simulink model "carsim_with_simulink14dof_random_control"  (R2023b)
settings: Solver=FixedStepAuto  StartTime=0.0  StopTime=25  FixedStep=0.001  RelTol=1e-3  EnableMultiTasking=on
values from neighbouring files (symbols this model uses):
  A = 5    [unlinear_vehicle_Parameters.m]
  Bf = 1.725    [unlinear_vehicle_Parameters.m]
  Br = 1.750    (= 1.75)    [unlinear_vehicle_Parameters.m]
  Cd = 0.4    [unlinear_vehicle_Parameters.m]
  Cs_f = 4302    [unlinear_vehicle_Parameters.m]
  f = 0.01    [unlinear_vehicle_Parameters.m]
  g = 9.8    [Truck_simulate.m]    (also in unlinear_vehicle_Parameters.m)
  He = 0.45    [unlinear_vehicle_Parameters.m]
  Hp = 0.2    [unlinear_vehicle_Parameters.m]
  I_tire = 0.7    [unlinear_vehicle_Parameters.m]
  Ix = 423.3    [unlinear_vehicle_Parameters.m]
  Iy = 1762.5    [unlinear_vehicle_Parameters.m]
  Iz = 1762.5    [unlinear_vehicle_Parameters.m]
  ks_f = 189000    [unlinear_vehicle_Parameters.m]
  kw = 220000    [unlinear_vehicle_Parameters.m]
  Lf = 1.330    (= 1.33)    [unlinear_vehicle_Parameters.m]
  Lr = 3.140 - 1.330    (= 1.81)    [unlinear_vehicle_Parameters.m]
  m = m_sprung + m_load + m_unsprung    (= 10505)    [Truck_simulate.m]    (also in unlinear_vehicle_Parameters.m = 1407.3)
  mb = 1128.5 + 000    (= 1128.5)    [unlinear_vehicle_Parameters.m]
  mw = 139.4 / 2    (= 69.7)    [unlinear_vehicle_Parameters.m]
  p = 1.206    [unlinear_vehicle_Parameters.m]
  r = 0.510    (= 0.51)    [Truck_simulate.m]    (also in unlinear_vehicle_Parameters.m = 0.287)
  vx0 = 5    [Truck_simulate.m]    (also in unlinear_vehicle_Parameters.m)
  vy0 = 0    [Truck_simulate.m]    (also in unlinear_vehicle_Parameters.m)
  w0 = vx0 / r    (= 9.80392156863)    [Truck_simulate.m]    (also in unlinear_vehicle_Parameters.m = 17.4216027875)
  wz0 = 0    [Truck_simulate.m]    (also in unlinear_vehicle_Parameters.m)
undefined symbols (not defined in the file or in its folder): Delta_act_seed, T_motor_seed
libraries: cstblocks x2, Solver_SF x1
(part 1 of 2)
settings Model: Creator=dzY  LastModifiedBy=Admin
settings SolverCC: AlgebraicLoopSolver=TrustRegion
settings DataIOCC: SaveFormat=Array  ReturnWorkspaceOutputs=off
settings OptimizationCC: LifeSpan=inf
settings DebuggingCC: SolverPrmCheckMsg=warning  UnconnectedInputMsg=warning  UnconnectedOutputMsg=warning  UnconnectedLineMsg=warning  SFUnexpectedBacktrackingDiag=warning  SFNoUnconditionalDefaultTransitionDiag=warning  SFExecutionAtInitializationDiag=none  ArithmeticOperatorsInVariantConditions=warning
settings HardwareCC: ProdBitPerPointer=32  ProdBitPerSizeT=32  ProdBitPerPtrDiffT=32  ProdLargestAtomicFloat=None  ProdIntDivRoundTo=Undefined  ProdEndianess=Unspecified  ProdWordSize=32  ProdHWDeviceType=32-bit Generic
settings ModelReferenceCC: EnableRefExpFcnMdlSchedulingChecks=on  PropagateSignalLabelsOutOfModel=off
settings SFSimCC: SimUseLocalCustomCode=off  CustomCodeUndefinedFunction=UseInterfaceOnly
settings RTWCC: RTWUseLocalCustomCode=off
settings CodeAppCC: StateflowObjectComments=on
settings GRTTargetCC: TargetLangStandard=C89/C90 (ANSI)
settings ConfigComp: CovMetricSettings=dw  CovSaveCumulativeToWorkspaceVar=on  CovSaveSingleToWorkspaceVar=on  CovExternalEMLEnable=off  CovSFcnEnable=off

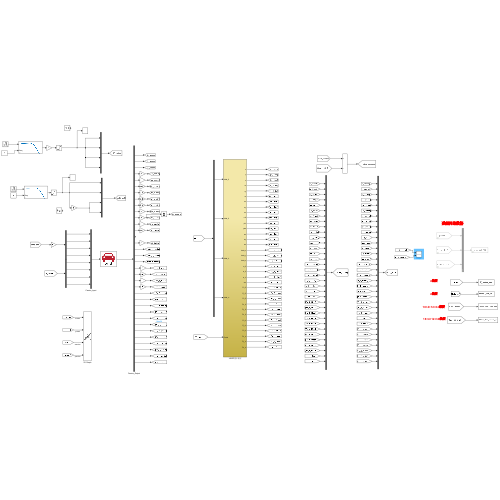
[thumbnail: Simulink's stored preview of the top-level diagram]
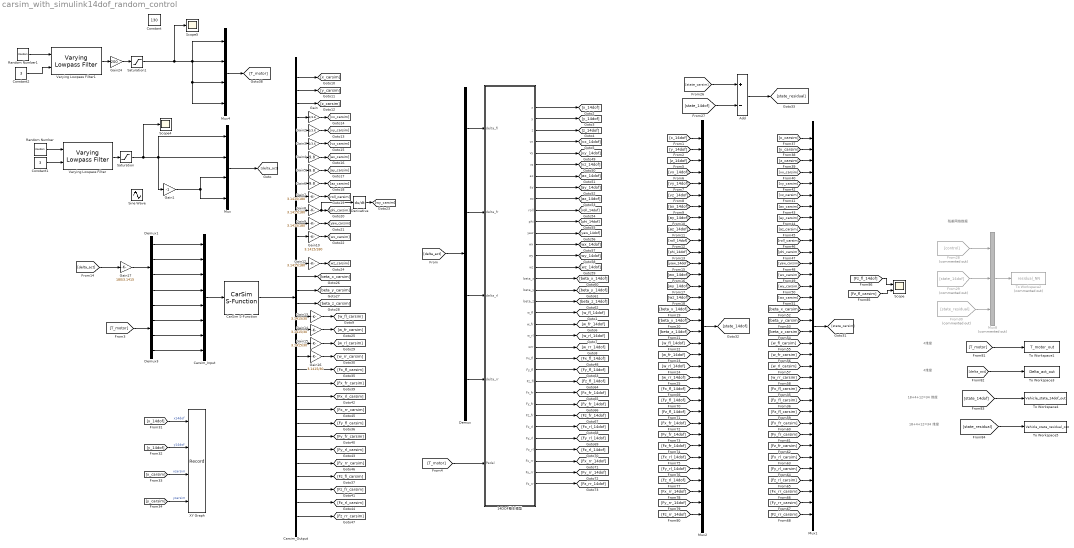
== system carsim_with_simulink14dof_random_control ==
  note: 4维度
  note: 残差网络数据
  note: 4维度
  note: 18+4+12=34维度
  note: 18+4+12=34维度
  14DOF整车模型 : Subsystem
  Add : Sum  Inputs=+-
  CarSim S-Function : Solver_SF/CarSim S-Function  Priority=1  SIMFILE=simfile.sim  Run_RTs=off  vs_state_ind=Run  StopMode_ind=Vehicle Model
  Carsim_Input : Mux  Inputs=8
  Carsim_Output : Demux  Outputs=34
  Constant : Constant  Value=130
  Constant1 : Constant  Value=3
  Constant2 : Constant  Value=3
  Demux : Demux
  Demux1 : Demux
  Demux3 : Demux
  Derivative : Derivative
  From28 : From  Commented=on  GotoTag=control
  From29 : From  Commented=on  GotoTag=state_14dof
  From30 : From  Commented=on  GotoTag=state_residual
  Gain : Gain  Gain=1/3.6
  Gain1 : Gain  Gain=-1
  Gain{7..10,12} (5 alike) : Gain  Gain=3.1415/180
  Gain{13..16} (4 alike) : Gain  Gain=3.1415/30
  Gain17 : Gain  Gain=180/3.1415
  Gain2 : Gain  Gain=1/3.6
  Gain24 : Gain  Gain=200
  Gain3 : Gain  Gain=1/3.6
  Gain4 : Gain  Gain=9.8
  Gain5 : Gain  Gain=9.8
  Gain6 : Gain  Gain=9.8
  Mux : Mux
  Mux1 : Mux  Inputs=34
  Mux2 : Mux  Inputs=34
  Mux4 : Mux
  Mux8 : Mux  Commented=on  Inputs=3
  Random Number : RandomNumber  Variance=20  Seed=Delta_act_seed  SampleTime=0.001
  Random Number1 : RandomNumber  Mean=0.1  Variance=50  Seed=T_motor_seed  SampleTime=0.001
  Saturation : Saturate  UpperLimit=0.35  LowerLimit=-0.35
  Saturation1 : Saturate  UpperLimit=150  LowerLimit=-150
  Scope : Scope  NumInputPorts=2
  Scope4 : Scope
  Scope5 : Scope
  Sine Wave : Sin  Amplitude=0.25  Frequency=0.4  SampleTime=0
  To Workspace1 : ToWorkspace  VariableName=T_motor_out  SaveFormat=Timeseries  SampleTime=-1
  To Workspace2 : ToWorkspace  Commented=on  VariableName=residual_NN  SaveFormat=Timeseries  SampleTime=-1
  To Workspace3 : ToWorkspace  VariableName=Delta_act_out  SaveFormat=Timeseries  SampleTime=-1
  To Workspace4 : ToWorkspace  VariableName=Vehicle_state_14dof_out  SaveFormat=Timeseries  SampleTime=-1
  To Workspace5 : ToWorkspace  VariableName=Vehicle_state_residual_out  SaveFormat=Timeseries  SampleTime=-1
  Varying Lowpass Filter : cstblocks/Linear Parameter Varying/Varying Lowpass Filter  N=8
  Varying Lowpass Filter1 : cstblocks/Linear Parameter Varying/Varying Lowpass Filter  N=8
  XY Graph : Record  RecordToFile=on  FileSettingsInternal="{\"entries\":[{\"content\":{\"excelSettings\":{\"content\":{},\"type\":\"Streamout.ExcelSettings\"}},\"type\":\"Streamout.FileSettingStorage\",\"uuid\":\"\"}],\"packageUris\":[\"http:\\/\\/schema.mathworks.com\\/mf0\\/streamout_blocks\\/R2020a\"],\"version\":\"1.0\"}"  Layout=[1 1]  SignalsInternal="{\"entries\":[{\"content\":{\"signals\":[{\"content\":{\"blockPath\":[],\"dimensions\":[1],\"domain\":\"\",\"lineColor\":\"#a2142f\",\"plots\":[1],\"port\":1,\"sid\":[\"\"],\"signalID\":3004,\"signalName\":\"x14dof\"},\"type\":\"RecordBlkView.Signal\",\"uuid\":\"\"},{\"content\":{\"blockPath\":[],\"dimensions\":[1],\"domain\":\"\",\"lineColor\":\"#139fff\",\"plots\":[1],\"port\":2,\"sid\":[\"\"],\"signalID\":3008,\"signalName\":\"y14dof\"},\"type\":\"RecordBlkView.Signal\",\"uuid\":\"\"},{\"content\":{\"blockPath\":[],\"dimensions\":[1],\"domain\":\"\",\"lineColor\":\"#77ac30\",\"plots\":[1],\"port\":3,\"sid\":[\"\"],\"signalID\":3012,\"signalName\":\"xcarsim\"},\"type\":\"RecordBlkView.Signal\",\"uuid\":\"\"},{\"content\":{\"blockPath\":[],\"dimensions\":[1],\"domain\":\"\",\"lineColor\":\"#4dbeee\",\"plots\":[1],\"port\":4,\"sid\":[\"\"],\"signalID\":3016,\"signalName\":\"ycarsim\"},\"type\":\"RecordBlkView.Signal\",\"uuid\":\"\"}]},\"type\":\"RecordBlkView.InputSignals\",\"uuid\":\"\"}],\"packageUris\":[\"http:\\/\\/schema.mathworks.com\\/mf0\\/streamout_blocks\\/R2020a\"],\"version\":\"1.0\"}"  VisualizationBindings="{\"xyplotplugin\":{\"info\":[{\"series\":[{\"bindingParametersList\":[{\"parameter\":\"X-Axis\",\"signalID\":3004,\"signalName\":\"x14dof\"},{\"parameter\":\"Y-Axis\",\"signalID\":3008,\"signalName\":\"y14dof\"}],\"seriesID\":21335},{\"bindingParametersList\":[{\"parameter\":\"X-Axis\",\"signalID\":3012,\"signalName\":\"xcarsim\"},{\"parameter\":\"Y-Axis\",\"signalID\":3016,\"signalName\":\"ycarsim\"}],\"seriesID\":24692}],\"subplotID\":1}]}}"  CompatibilityTag=XY
  wires:
  [T_motor] -> 14DOF整车模型/5(Pedal)
  Mux4/1 -> [T_motor]
  Saturation1/1 -> Mux4/1, Mux4/4, Mux4/3, Mux4/2, Scope5/1
  Carsim_Input/1 -> CarSim S-Function/1
  CarSim S-Function/1 -> Carsim_Output/1
  [T_motor] -> Demux3/1
  Demux3/1 -> Carsim_Input/5
  Demux3/2 -> Carsim_Input/6
  Demux3/3 -> Carsim_Input/7
  Demux3/4 -> Carsim_Input/8
  14DOF整车模型/1(x) -> [x_14dof]
  14DOF整车模型/2(y) -> [y_14dof]
  14DOF整车模型/3(z) -> [z_14dof]
  14DOF整车模型/4(vx) -> [vx_14dof]
  14DOF整车模型/5(vy) -> [vy_14dof]
  14DOF整车模型/6(vz) -> [vz_14dof]
  14DOF整车模型/7(ax) -> [ax_14dof]
  14DOF整车模型/8(ay) -> [ay_14dof]
  14DOF整车模型/9(az) -> [az_14dof]
  14DOF整车模型/10(roll) -> [roll_14dof]
  14DOF整车模型/11(phi) -> [phi_14dof]
  14DOF整车模型/12(yaw) -> [yaw_14dof]
  14DOF整车模型/13(wx) -> [wx_14dof]
  14DOF整车模型/14(wy) -> [wy_14dof]
  14DOF整车模型/15(wz) -> [wz_14dof]
  14DOF整车模型/16(beta_x) -> [beta_x_14dof]
  14DOF整车模型/17(beta_y) -> [beta_y_14dof]
  14DOF整车模型/18(beta_z) -> [beta_z_14dof]
  [x_14dof] -> Mux2/1
  [y_14dof] -> Mux2/2
  [z_14dof] -> Mux2/3
  [vx_14dof] -> Mux2/4
  [vy_14dof] -> Mux2/5
  [vz_14dof] -> Mux2/6
  [ax_14dof] -> Mux2/7
  [ay_14dof] -> Mux2/8
  [az_14dof] -> Mux2/9
  [roll_14dof] -> Mux2/10
  [phi_14dof] -> Mux2/11
  [yaw_14dof] -> Mux2/12
  [wx_14dof] -> Mux2/13
  [wy_14dof] -> Mux2/14
  [wz_14dof] -> Mux2/15
  [beta_x_14dof] -> Mux2/16
  [beta_y_14dof] -> Mux2/17
  [beta_z_14dof] -> Mux2/18
  Mux2/1 -> [state_14dof]
  Saturation/1 -> Mux/1, Mux/2, Gain1/1, Scope4/1
  Mux/1 -> [delta_act]
  Gain1/1 -> Mux/4, Mux/3
  Demux/4 -> 14DOF整车模型/4(delta_rr)
  Demux/3 -> 14DOF整车模型/3(delta_rl)
  Demux/2 -> 14DOF整车模型/2(delta_fr)
  Demux/1 -> 14DOF整车模型/1(delta_fl)
  [delta_act] -> Demux/1
  Demux1/4 -> Carsim_Input/4
  Demux1/3 -> Carsim_Input/3
  Demux1/2 -> Carsim_Input/2
  Demux1/1 -> Carsim_Input/1
  14DOF整车模型/19(w_fl) -> [w_fl_14dof]
  14DOF整车模型/20(w_fr) -> [w_fr_14dof]
  14DOF整车模型/21(w_rl) -> [w_rl_14dof]
  14DOF整车模型/22(wrr) -> [w_rr_14dof]
  [w_fl_14dof] -> Mux2/19
  [w_fr_14dof] -> Mux2/20
  [w_rl_14dof] -> Mux2/21
  [w_rr_14dof] -> Mux2/22
  Carsim_Output/2 -> [y_carsim]
  Carsim_Output/1 -> [x_carsim]
  Carsim_Output/3 -> [z_carsim]
  Carsim_Output/16 -> [beta_x_carsim]
  Carsim_Output/17 -> [beta_y_carsim]
  Carsim_Output/18 -> [beta_z_carsim]
  [state_14dof] -> Add/2
  [state_carsim] -> Add/1
  Add/1 -> [state_residual]
  Mux8/1 -> To Workspace2/1
  From28/1 -> Mux8/1
  From29/1 -> Mux8/2
  From30/1 -> Mux8/3
  Carsim_Output/6 -> Gain3/1
  Gain3/1 -> [vz_carsim]
  Carsim_Output/5 -> Gain2/1
  Gain2/1 -> [vy_carsim]
  Gain/1 -> [vx_carsim]
  Carsim_Output/4 -> Gain/1
  Carsim_Output/7 -> Gain4/1
  Gain4/1 -> [ax_carsim]
  Carsim_Output/8 -> Gain5/1
  Gain5/1 -> [ay_carsim]
  Carsim_Output/9 -> Gain6/1
  Gain6/1 -> [az_carsim]
  Carsim_Output/10 -> Gain7/1
  Gain7/1 -> [roll_carsim]
  Carsim_Output/11 -> Gain8/1
  Gain8/1 -> Derivative/1, [phi_carsim]
  Carsim_Output/12 -> Gain9/1
  Gain9/1 -> [yaw_carsim]
  Carsim_Output/15 -> Gain12/1
  Carsim_Output/13 -> Gain10/1
  Gain10/1 -> [wx_carsim]
  Gain12/1 -> [wz_carsim]
  Carsim_Output/19 -> Gain13/1
  Gain13/1 -> [w_fl_carsim]
  Carsim_Output/20 -> Gain14/1
  Gain14/1 -> [w_fr_carsim]
  Carsim_Output/21 -> Gain15/1
  Carsim_Output/22 -> Gain16/1
  Gain15/1 -> [w_rl_carsim]
  Gain16/1 -> [w_rr_carsim]
  Gain17/1 -> Demux1/1
  [delta_act] -> Gain17/1
  Derivative/1 -> [wy_carsim]
  [x_carsim] -> Mux1/1
  [y_carsim] -> Mux1/2
  [z_carsim] -> Mux1/3
  [vx_carsim] -> Mux1/4
  [vy_carsim] -> Mux1/5
  [vz_carsim] -> Mux1/6
  [ax_carsim] -> Mux1/7
  [ay_carsim] -> Mux1/8
  [az_carsim] -> Mux1/9
  [roll_carsim] -> Mux1/10
  [phi_carsim] -> Mux1/11
  [yaw_carsim] -> Mux1/12
  [wx_carsim] -> Mux1/13
  [wy_carsim] -> Mux1/14
  [wz_carsim] -> Mux1/15
  [beta_x_carsim] -> Mux1/16
  [beta_y_carsim] -> Mux1/17
  [beta_z_carsim] -> Mux1/18
  [w_fl_carsim] -> Mux1/19
  [w_fr_carsim] -> Mux1/20
  [w_rl_carsim] -> Mux1/21
  [w_rr_carsim] -> Mux1/22
  Mux1/1 -> [state_carsim]
  Constant2/1 -> Varying Lowpass Filter1/2
  Random Number1/1 -> Varying Lowpass Filter1/1
  Gain24/1 -> Saturation1/1
  Varying Lowpass Filter1/1 -> Gain24/1
  Random Number/1 -> Varying Lowpass Filter/1
  Constant1/1 -> Varying Lowpass Filter/2
  Varying Lowpass Filter/1 -> Saturation/1
  [x_14dof] -> XY Graph/1  "x14dof"
  [x_carsim] -> XY Graph/3  "xcarsim"
  [y_carsim] -> XY Graph/4  "ycarsim"
  [y_14dof] -> XY Graph/2  "y14dof"
  [Fx_fl_carsim] -> Mux1/23
  [Fy_fl_carsim] -> Mux1/24
  [Fz_fl_carsim] -> Mux1/25
  [Fx_fr_carsim] -> Mux1/26
  [Fy_fr_carsim] -> Mux1/27
  [Fz_fr_carsim] -> Mux1/28
  [Fx_rl_carsim] -> Mux1/29
  [Fy_rl_carsim] -> Mux1/30
  [Fz_rl_carsim] -> Mux1/31
  [Fx_rr_carsim] -> Mux1/32
  [Fy_rr_carsim] -> Mux1/33
  [Fz_rr_carsim] -> Mux1/34
  14DOF整车模型/23(Fx_fl) -> [Fx_fl_14dof]
  14DOF整车模型/24(Fy_fl) -> [Fy_fl_14dof]
  14DOF整车模型/25(Fz_fl) -> [Fz_fl_14dof]
  14DOF整车模型/26(Fx_fr) -> [Fx_fr_14dof]
  14DOF整车模型/27(Fy_fr) -> [Fy_fr_14dof]
  14DOF整车模型/28(Fz_fr) -> [Fz_fr_14dof]
  14DOF整车模型/29(Fx_rl) -> [Fx_rl_14dof]
  14DOF整车模型/30(Fy_rl) -> [Fy_rl_14dof]
  14DOF整车模型/31(Fz_rl) -> [Fz_rl_14dof]
  14DOF整车模型/32(Fx_rr) -> [Fx_rr_14dof]
  14DOF整车模型/33(Fy_rr) -> [Fy_rr_14dof]
  14DOF整车模型/34(Fz_rr) -> [Fz_rr_14dof]
  [Fx_fl_14dof] -> Mux2/23
  [Fy_fl_14dof] -> Mux2/24
  [Fz_fl_14dof] -> Mux2/25
  [Fx_fr_14dof] -> Mux2/26
  [Fy_fr_14dof] -> Mux2/27
  [Fz_fr_14dof] -> Mux2/28
  [Fx_rl_14dof] -> Mux2/29
  [Fy_rl_14dof] -> Mux2/30
  [Fz_rl_14dof] -> Mux2/31
  [Fx_rr_14dof] -> Mux2/32
  [Fy_rr_14dof] -> Mux2/33
  [Fz_rr_14dof] -> Mux2/34
  [T_motor] -> To Workspace1/1
  [delta_act] -> To Workspace3/1
  [state_14dof] -> To Workspace4/1
  [state_residual] -> To Workspace5/1
  [Fz_fl_14dof] -> Scope/1
  [Fz_fl_carsim] -> Scope/2
  Carsim_Output/23 -> [Fx_fl_carsim]
  Carsim_Output/24 -> [Fx_fr_carsim]
  Carsim_Output/25 -> [Fx_rl_carsim]
  Carsim_Output/26 -> [Fx_rr_carsim]
  Carsim_Output/27 -> [Fy_fl_carsim]
  Carsim_Output/28 -> [Fy_fr_carsim]
  Carsim_Output/29 -> [Fy_rl_carsim]
  Carsim_Output/30 -> [Fy_rr_carsim]
  Carsim_Output/31 -> [Fz_fl_carsim]
  Carsim_Output/32 -> [Fz_fr_carsim]
  Carsim_Output/33 -> [Fz_rl_carsim]
  Carsim_Output/34 -> [Fz_rr_carsim]

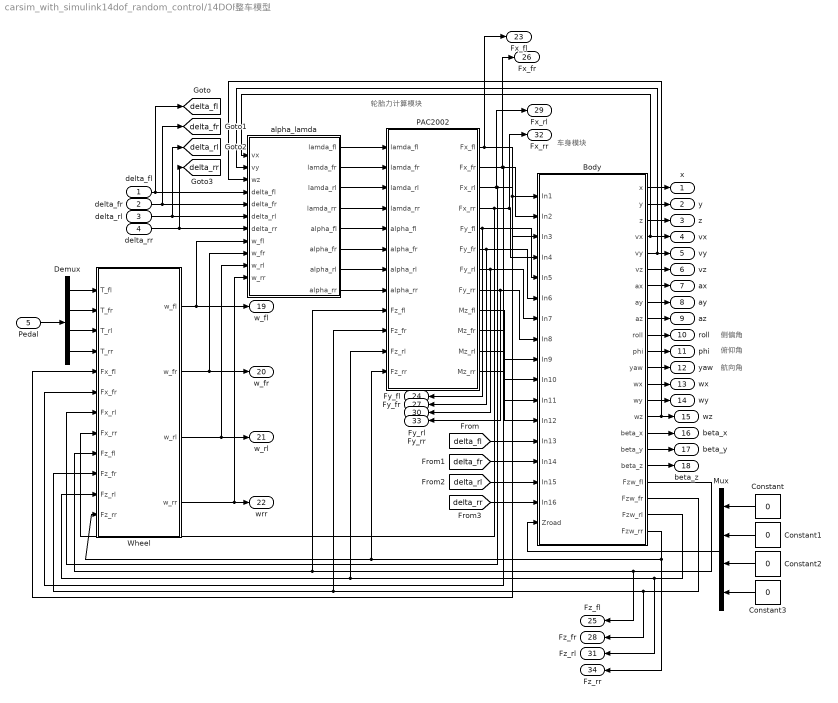
== system carsim_with_simulink14dof_random_control/14DOF整车模型 ==
  note: 车身模块
  note: 航向角
  note: 侧偏角
  note: 俯仰角
  note: 轮胎力计算模块
  delta_fl : Inport
  delta_fr : Inport  Port=2
  delta_rl : Inport  Port=3
  delta_rr : Inport  Port=4
  Pedal : Inport  Port=5
  Body : Subsystem
  Constant{,1..3} (4 alike) : Constant  Value=0
  Demux : Demux
  Mux : Mux
  PAC2002 : Subsystem
  Wheel : Subsystem
  alpha_lamda : Subsystem
  x : Outport
  y : Outport  Port=2
  z : Outport  Port=3
  vx : Outport  Port=4
  vy : Outport  Port=5
  vz : Outport  Port=6
  ax : Outport  Port=7
  ay : Outport  Port=8
  az : Outport  Port=9
  roll : Outport  Port=10
  phi : Outport  Port=11
  yaw : Outport  Port=12
  wx : Outport  Port=13
  wy : Outport  Port=14
  wz : Outport  Port=15
  beta_x : Outport  Port=16
  beta_y : Outport  Port=17
  beta_z : Outport  Port=18
  w_fl : Outport  Port=19
  w_fr : Outport  Port=20
  w_rl : Outport  Port=21
  wrr : Outport  Port=22
  Fx_fl : Outport  Port=23
  Fy_fl : Outport  Port=24
  Fz_fl : Outport  Port=25
  Fx_fr : Outport  Port=26
  Fy_fr : Outport  Port=27
  Fz_fr : Outport  Port=28
  Fx_rl : Outport  Port=29
  Fy_rl : Outport  Port=30
  Fz_rl : Outport  Port=31
  Fx_rr : Outport  Port=32
  Fy_rr : Outport  Port=33
  Fz_rr : Outport  Port=34
  tag scope: delta_fl=global, delta_fr=global, delta_rl=global, delta_rr=global
  wires:
  delta_fl/1 -> alpha_lamda/4(delta_fl), [delta_fl]
  delta_rr/1 -> alpha_lamda/7(delta_rr), [delta_rr]
  delta_fr/1 -> alpha_lamda/5(delta_fr), [delta_fr]
  delta_rl/1 -> [delta_rl], alpha_lamda/6(delta_rl)
  alpha_lamda/1(lamda_fl) -> PAC2002/1(lamda_fl)
  alpha_lamda/7(alpha_rl) -> PAC2002/7(alpha_rl)
  Wheel/2(w_fr) -> w_fr/1, alpha_lamda/9(w_fr)
  PAC2002/5(Fy_fl) -> Body/5(In5), Fy_fl/1
  alpha_lamda/2(lamda_fr) -> PAC2002/2(lamda_fr)
  alpha_lamda/5(alpha_fl) -> PAC2002/5(alpha_fl)
  alpha_lamda/3(lamda_rl) -> PAC2002/3(lamda_rl)
  alpha_lamda/4(lamda_rr) -> PAC2002/4(lamda_rr)
  PAC2002/9(Mz_fl) -> Body/9(In9)
  PAC2002/10(Mz_fr) -> Body/10(In10)
  Wheel/4(w_rr) -> alpha_lamda/11(w_rr), wrr/1
  PAC2002/4(Fx_rr) -> Fx_rr/1, Body/4(In4), Wheel/8(Fx_rr)
  alpha_lamda/6(alpha_fr) -> PAC2002/6(alpha_fr)
  PAC2002/3(Fx_rl) -> Fx_rl/1, Body/3(In3), Wheel/7(Fx_rl)
  Wheel/3(w_rl) -> w_rl/1, alpha_lamda/10(w_rl)
  PAC2002/7(Fy_rl) -> Fy_rl/1, Body/7(In7)
  PAC2002/2(Fx_fr) -> Body/2(In2), Wheel/6(Fx_fr), Fx_fr/1
  PAC2002/8(Fy_rr) -> Fy_rr/1, Body/8(In8)
  alpha_lamda/8(alpha_rr) -> PAC2002/8(alpha_rr)
  PAC2002/1(Fx_fl) -> Wheel/5(Fx_fl), Body/1(In1), Fx_fl/1
  PAC2002/12(Mz_rr) -> Body/12(In12)
  Demux/3 -> Wheel/3(T_rl)
  Demux/2 -> Wheel/2(T_fr)
  Demux/1 -> Wheel/1(T_fl)
  PAC2002/11(Mz_rl) -> Body/11(In11)
  Demux/4 -> Wheel/4(T_rr)
  PAC2002/6(Fy_fr) -> Fy_fr/1, Body/6(In6)
  Pedal/1 -> Demux/1
  [delta_fl] -> Body/13(In13)
  [delta_fr] -> Body/14(In14)
  [delta_rl] -> Body/15(In15)
  [delta_rr] -> Body/16(In16)
  Mux/1 -> Body/17(Zroad)
  Body/1(x) -> x/1
  Body/2(y) -> y/1
  Body/3(z) -> z/1
  Body/4(vx) -> vx/1, alpha_lamda/1(vx)
  Body/5(vy) -> alpha_lamda/2(vy), vy/1
  Body/6(vz) -> vz/1
  Body/7(ax) -> ax/1
  Body/8(ay) -> ay/1
  Body/9(az) -> az/1
  Body/10(roll) -> roll/1
  Body/11(phi) -> phi/1
  Body/12(yaw) -> yaw/1
  Body/13(wx) -> wx/1
  Body/16(beta_x) -> beta_x/1
  Body/14(wy) -> wy/1
  Body/15(wz) -> alpha_lamda/3(wz), wz/1
  Body/18(beta_z) -> beta_z/1
  Body/19(Fzw_fl) -> Fz_fl/1, PAC2002/9(Fz_fl), Wheel/9(Fz_fl)
  Body/20(Fzw_fr) -> Fz_fr/1, PAC2002/10(Fz_fr), Wheel/10(Fz_fr)
  Body/21(Fzw_rl) -> Fz_rl/1, Wheel/11(Fz_rl), PAC2002/11(Fz_rl)
  Body/22(Fzw_rr) -> Fz_rr/1, PAC2002/12(Fz_rr), Wheel/12(Fz_rr)
  Wheel/1(w_fl) -> w_fl/1, alpha_lamda/8(w_fl)
  Body/17(beta_y) -> beta_y/1
  Constant/1 -> Mux/1
  Constant1/1 -> Mux/2
  Constant2/1 -> Mux/3
  Constant3/1 -> Mux/4

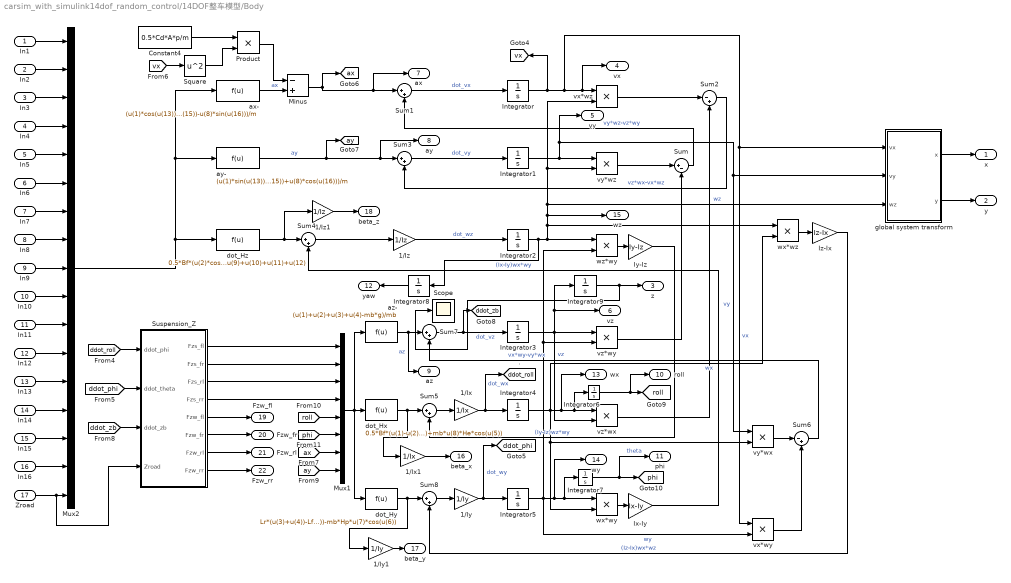
== system carsim_with_simulink14dof_random_control/14DOF整车模型/Body ==
  In1 : Inport
  In2 : Inport  Port=2
  In3 : Inport  Port=3
  In4 : Inport  Port=4
  In5 : Inport  Port=5
  In6 : Inport  Port=6
  In7 : Inport  Port=7
  In8 : Inport  Port=8
  In9 : Inport  Port=9
  In10 : Inport  Port=10
  In11 : Inport  Port=11
  In12 : Inport  Port=12
  In13 : Inport  Port=13
  In14 : Inport  Port=14
  In15 : Inport  Port=15
  In16 : Inport  Port=16
  Zroad : Inport  Port=17
  1/Ix : Gain  Gain=1/Ix
  1/Ix1 : Gain  Gain=1/Ix
  1/Iy : Gain  Gain=1/Iy
  1/Iy1 : Gain  Gain=1/Iy
  1/Iz : Gain  Gain=1/Iz
  1/Iz1 : Gain  Gain=1/Iz
  Constant4 : Constant  Value=0.5*Cd*A*p/m
  Integrator : Integrator  InitialCondition=vx0  LimitOutput=on  LowerSaturationLimit=0
  Integrator1 : Integrator  InitialCondition=vy0
  Integrator2 : Integrator  InitialCondition=wz0
  Integrator{3..6,8} (5 alike) : Integrator
  Integrator7 : Integrator  InitialCondition=1.2245e-3
  Integrator9 : Integrator  InitialCondition=-0.131
  Ix-Iy : Gain  Gain=Ix-Iy
  Iy-Iz : Gain  Gain=Iy-Iz
  Iz-Ix : Gain  Gain=Iz-Ix
  Minus : Sum  Inputs=-+
  Mux1 : Mux  Inputs=8
  Mux2 : Mux  Inputs=17
  Product : Product
  Scope : Scope
  Square : Math  Operator=square
  Sum : Sum  Inputs=|+-
  Sum{1,3..5,7..8} (6 alike) : Sum  Inputs=|++
  Sum2 : Sum  Inputs=|-+
  Sum6 : Sum  Inputs=|-+
  Suspension_Z : Subsystem
  ax- : Fcn  Expr="(u(1)*cos(u(13))+u(2)*cos(u(14))-u(5)*sin(u(13))-u(6)*sin(u(14))+   u(3)*cos(u(15))+u(4)*cos(u(16))-u(7)*sin(u(15))-u(8)*sin(u(16)))/m"
  ay- : Fcn  Expr=(u(1)*sin(u(13))+u(2)*sin(u(14))+u(5)*cos(u(13))+u(6)*cos(u(14))+u(3)*sin(u(15))+u(4)*sin(u(16))+u(7)*cos(u(15))+u(8)*cos(u(16)))/m
  az- : Fcn  Expr=(u(1)+u(2)+u(3)+u(4)-mb*g)/mb
  dot_Hx : Fcn  Expr=0.5*Bf*(u(1)-u(2))+0.5*Br*(u(3)-u(4))+mb*g*He*sin(u(5))+mb*u(8)*He*cos(u(5))
  dot_Hy : Fcn  Expr=Lr*(u(3)+u(4))-Lf*(u(1)+u(2))+mb*g*Hp*sin(u(6))-mb*Hp*u(7)*cos(u(6))
  dot_Hz : Fcn  Expr=0.5*Bf*(u(2)*cos(u(14))-u(1)*cos(u(13))-u(6)*sin(u(14))+u(5)*sin(u(13)))+0.5*Br*(u(4)*cos(u(16))-u(3)*cos(u(15))-u(8)*sin(u(16))+u(7)*sin(u(15)))+Lf*(u(1)*sin(u(13))+u(5)*cos(u(13))+u(2)*sin(u(14))+u(6)*cos(u(14)))-Lr*(u(3)*sin(u(15))+u(7)*cos(u(15))+u(4)*sin(u(16))+u(8)*cos(u(16)))+u(9)+u(10)+u(11)+u(12)
  global system transform : Subsystem
  vx*wy : Product
  vx*wz : Product
  vy*wx : Product
  vy*wz : Product
  vz*wx : Product
  vz*wy : Product
  wx*wy : Product
  wx*wz : Product
  wz*wy : Product
  x : Outport
  y : Outport  Port=2
  z : Outport  Port=3
  vx : Outport  Port=4
  vy : Outport  Port=5
  vz : Outport  Port=6
  ax : Outport  Port=7
  ay : Outport  Port=8
  az : Outport  Port=9
  roll : Outport  Port=10
  phi : Outport  Port=11
  yaw : Outport  Port=12
  wx : Outport  Port=13
  wy : Outport  Port=14
  wz : Outport  Port=15
  beta_x : Outport  Port=16
  beta_y : Outport  Port=17
  beta_z : Outport  Port=18
  Fzw_fl : Outport  Port=19
  Fzw_fr : Outport  Port=20
  Fzw_rl : Outport  Port=21
  Fzw_rr : Outport  Port=22
  tag scope: ax=global, ay=global, ddot_phi=global, ddot_roll=global, ddot_zb=global, phi=global, roll=global, vx=global
  wires:
  ay-/1 -> [ay], ay/1, Sum3/1  "ay"
  vx*wz/1 -> Sum2/1
  Integrator/1 -> vx*wy/1, global system transform/1(vx), vx/1, vx*wz/1, [vx]  "vx"
  Suspension_Z/3(Fzs_rl) -> Mux1/3
  [phi] -> Mux1/6
  vy*wx/1 -> Sum6/1
  wz*wy/1 -> Iy-Iz/1
  vy*wz/1 -> Sum/1
  Integrator5/1 -> wy/1, wx*wy/1, Integrator7/1, wz*wy/2, vz*wy/2, vx*wy/2  "wy"
  Sum7/1 -> Integrator3/1, [ddot_zb]  "dot_vz"
  Integrator2/1 -> Integrator8/1, wz*wy/1, wz/1, vx*wz/2, vy*wz/2, global system transform/3(wz), wx*wz/1  "wz"
  az-/1 -> Sum7/1, az/1  "az"
  dot_Hz/1 -> 1/Iz1/1, Sum4/1
  vx*wy/1 -> Sum6/2
  vz*wx/1 -> Sum2/2
  Integrator3/1 -> vz*wy/1, vz*wx/2, vz/1, Integrator9/1  "vz"
  Mux1/1 -> az-/1, dot_Hx/1, dot_Hy/1
  Minus/1 -> ax/1, Sum1/1, [ax]
  dot_Hy/1 -> 1/Iy1/1, Sum8/1
  Mux2/1 -> ax-/1, ay-/1, dot_Hz/1
  In5/1 -> Mux2/5
  global system transform/1(x) -> x/1
  [ddot_roll] -> Suspension_Z/1(ddot_phi)
  Integrator1/1 -> vy*wz/1, vy/1, vy*wx/1, global system transform/2(vy)  "vy"
  Suspension_Z/7(Fzw_rl) -> Fzw_rl/1
  1/Ix/1 -> Integrator4/1, [ddot_roll]  "dot_wx"
  1/Iy/1 -> Integrator5/1, [ddot_phi]  "dot_wy"
  wx*wy/1 -> Ix-Iy/1
  Integrator7/1 -> phi/1, [phi]  "theta"
  Square/1 -> Product/2
  1/Iz/1 -> Integrator2/1  "dot_wz"
  Sum/1 -> Sum1/2  "vy*wz-vz*wy"
  Zroad/1 -> Suspension_Z/4(Zroad), Mux2/17
  Integrator4/1 -> wx/1, vz*wx/1, Integrator6/1, wx*wy/2, vy*wx/2, wx*wz/2  "wx"
  Sum2/1 -> Sum3/2  "vz*wx-vx*wz"
  Suspension_Z/6(Fzw_fr) -> Fzw_fr/1
  In12/1 -> Mux2/12
  Sum3/1 -> Integrator1/1  "dot_vy"
  wx*wz/1 -> Iz-Ix/1
  Sum6/1 -> Sum7/2  "vx*wy-vy*wx"
  In16/1 -> Mux2/16
  [ay] -> Mux1/8
  [vx] -> Square/1
  [ddot_zb] -> Suspension_Z/3(ddot_zb)
  Product/1 -> Minus/1
  Ix-Iy/1 -> Sum4/2  "(Ix-Iy)wx*wy"
  In2/1 -> Mux2/2
  Iz-Ix/1 -> Sum8/2  "(Iz-Ix)wx*wz"
  Sum4/1 -> 1/Iz/1
  Suspension_Z/2(Fzs_fr) -> Mux1/2
  Integrator6/1 -> roll/1, [roll]
  Sum5/1 -> 1/Ix/1
  dot_Hx/1 -> 1/Ix1/1, Sum5/1
  Sum8/1 -> 1/Iy/1
  ax-/1 -> Minus/2  "ax"
  Iy-Iz/1 -> Sum5/2  "(Iy-Iz)wz*wy"
  [ddot_phi] -> Suspension_Z/2(ddot_theta)
  Constant4/1 -> Product/1
  vz*wy/1 -> Sum/2
  Suspension_Z/4(Fzs_rr) -> Mux1/4
  In6/1 -> Mux2/6
  [roll] -> Mux1/5
  Suspension_Z/1(Fzs_fl) -> Mux1/1
  Sum1/1 -> Integrator/1  "dot_vx"
  Suspension_Z/8(Fzw_rr) -> Fzw_rr/1
  [ax] -> Mux1/7
  In14/1 -> Mux2/14
  In11/1 -> Mux2/11
  In3/1 -> Mux2/3
  Suspension_Z/5(Fzw_fl) -> Fzw_fl/1
  Integrator8/1 -> yaw/1
  In1/1 -> Mux2/1
  In10/1 -> Mux2/10
  In4/1 -> Mux2/4
  In15/1 -> Mux2/15
  global system transform/2(y) -> y/1
  Integrator9/1 -> Scope/1, z/1
  In8/1 -> Mux2/8
  In13/1 -> Mux2/13
  In9/1 -> Mux2/9
  In7/1 -> Mux2/7
  1/Iz1/1 -> beta_z/1
  1/Ix1/1 -> beta_x/1
  1/Iy1/1 -> beta_y/1

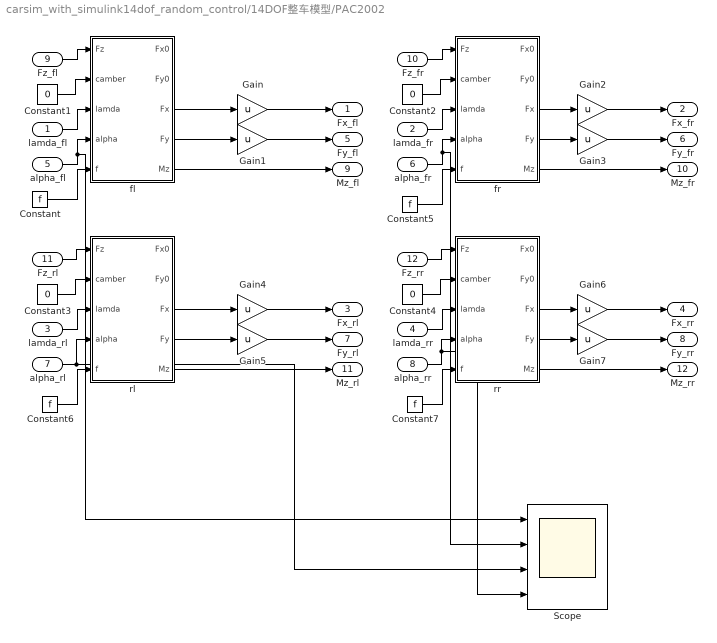
== system carsim_with_simulink14dof_random_control/14DOF整车模型/PAC2002 ==
  lamda_fl : Inport
  lamda_fr : Inport  Port=2
  lamda_rl : Inport  Port=3
  lamda_rr : Inport  Port=4
  alpha_fl : Inport  Port=5
  alpha_fr : Inport  Port=6
  alpha_rl : Inport  Port=7
  alpha_rr : Inport  Port=8
  Fz_fl : Inport  Port=9
  Fz_fr : Inport  Port=10
  Fz_rl : Inport  Port=11
  Fz_rr : Inport  Port=12
  Constant{,5..7} (4 alike) : Constant  Value=f
  Constant{1..4} (4 alike) : Constant  Value=0
  Gain{,1..7} (8 alike) : Gain  Gain=u
  Scope : Scope  NumInputPorts=4
  fl : MATLAB Function  TreatAsAtomicUnit=on
  fr : MATLAB Function  TreatAsAtomicUnit=on
  rl : MATLAB Function  TreatAsAtomicUnit=on
  rr : MATLAB Function  TreatAsAtomicUnit=on
  Fx_fl : Outport
  Fx_fr : Outport  Port=2
  Fx_rl : Outport  Port=3
  Fx_rr : Outport  Port=4
  Fy_fl : Outport  Port=5
  Fy_fr : Outport  Port=6
  Fy_rl : Outport  Port=7
  Fy_rr : Outport  Port=8
  Mz_fl : Outport  Port=9
  Mz_fr : Outport  Port=10
  Mz_rl : Outport  Port=11
  Mz_rr : Outport  Port=12
  wires:
  Constant4/1 -> rr/2(camber)
  Constant3/1 -> rl/2(camber)
  Constant2/1 -> fr/2(camber)
  rr/5(Mz) -> Mz_rr/1
  rl/5(Mz) -> Mz_rl/1
  Fz_rr/1 -> rr/1(Fz)
  alpha_rr/1 -> Scope/4, rr/4(alpha)
  lamda_rr/1 -> rr/3(lamda)
  Fz_rl/1 -> rl/1(Fz)
  alpha_rl/1 -> Scope/3, rl/4(alpha)
  lamda_rl/1 -> rl/3(lamda)
  fr/5(Mz) -> Mz_fr/1
  Fz_fr/1 -> fr/1(Fz)
  alpha_fr/1 -> Scope/2, fr/4(alpha)
  lamda_fr/1 -> fr/3(lamda)
  fl/5(Mz) -> Mz_fl/1
  Constant1/1 -> fl/2(camber)
  Fz_fl/1 -> fl/1(Fz)
  alpha_fl/1 -> Scope/1, fl/4(alpha)
  lamda_fl/1 -> fl/3(lamda)
  fl/3(Fx) -> Gain/1
  fl/4(Fy) -> Gain1/1
  fr/4(Fy) -> Gain3/1
  rr/3(Fx) -> Gain6/1
  rr/4(Fy) -> Gain7/1
  rl/3(Fx) -> Gain4/1
  rl/4(Fy) -> Gain5/1
  fr/3(Fx) -> Gain2/1
  Gain/1 -> Fx_fl/1
  Gain1/1 -> Fy_fl/1
  Gain2/1 -> Fx_fr/1
  Gain3/1 -> Fy_fr/1
  Gain4/1 -> Fx_rl/1
  Gain5/1 -> Fy_rl/1
  Gain6/1 -> Fx_rr/1
  Gain7/1 -> Fy_rr/1
  Constant/1 -> fl/5(f)
  Constant5/1 -> fr/5(f)
  Constant6/1 -> rl/5(f)
  Constant7/1 -> rr/5(f)

== system carsim_with_simulink14dof_random_control/14DOF整车模型/Wheel ==
  T_fl : Inport
  T_fr : Inport  Port=2
  T_rl : Inport  Port=3
  T_rr : Inport  Port=4
  Fx_fl : Inport  Port=5
  Fx_fr : Inport  Port=6
  Fx_rl : Inport  Port=7
  Fx_rr : Inport  Port=8
  Fz_fl : Inport  Port=9
  Fz_fr : Inport  Port=10
  Fz_rl : Inport  Port=11
  Fz_rr : Inport  Port=12
  fl : Subsystem
  fr : Subsystem
  rl : Subsystem
  rr : Subsystem
  w_fl : Outport
  w_fr : Outport  Port=2
  w_rl : Outport  Port=3
  w_rr : Outport  Port=4
  wires:
  rr/1(w_rr) -> w_rr/1
  Fz_rr/1 -> rr/3(Fz_rr)
  Fx_rr/1 -> rr/2(Fx_rr)
  T_rr/1 -> rr/1(T_rr)
  rl/1(w_rl) -> w_rl/1
  Fz_rl/1 -> rl/3(Fz_rl)
  Fx_rl/1 -> rl/2(Fx_rl)
  T_rl/1 -> rl/1(T_rl)
  Fz_fr/1 -> fr/3(Fz_fr)
  Fx_fr/1 -> fr/2(Fx_fr)
  T_fr/1 -> fr/1(T_fr)
  fr/1(w_fr) -> w_fr/1
  fl/1(w_fl) -> w_fl/1
  Fz_fl/1 -> fl/3(Fz_fl)
  Fx_fl/1 -> fl/2(Fx_fl)
  T_fl/1 -> fl/1(T_fl)

== system carsim_with_simulink14dof_random_control/14DOF整车模型/alpha_lamda ==
  vx : Inport
  vy : Inport  Port=2
  wz : Inport  Port=3
  delta_fl : Inport  Port=4
  delta_fr : Inport  Port=5
  delta_rl : Inport  Port=6
  delta_rr : Inport  Port=7
  w_fl : Inport  Port=8
  w_fr : Inport  Port=9
  w_rl : Inport  Port=10
  w_rr : Inport  Port=11
  alpha : Subsystem
  lamda : Subsystem
  lamda_fl : Outport
  lamda_fr : Outport  Port=2
  lamda_rl : Outport  Port=3
  lamda_rr : Outport  Port=4
  alpha_fl : Outport  Port=5
  alpha_fr : Outport  Port=6
  alpha_rl : Outport  Port=7
  alpha_rr : Outport  Port=8
  wires:
  alpha/1(alpha_fl) -> alpha_fl/1
  alpha/2(alpha_fr) -> alpha_fr/1
  alpha/3(alpha_rl) -> alpha_rl/1
  alpha/4(alpha_rr) -> alpha_rr/1
  vx/1 -> lamda/1(vx), alpha/1(vx)
  vy/1 -> lamda/2(vy), alpha/2(vy)
  wz/1 -> lamda/3(wz), alpha/3(wz)
  delta_fl/1 -> lamda/4(delta_fl), alpha/4(delta_fl)
  delta_fr/1 -> lamda/5(delta_fr), alpha/5(delta_fr)
  w_fl/1 -> lamda/6(w_fl)
  w_fr/1 -> lamda/7(w_fr)
  w_rl/1 -> lamda/8(w_rl)
  w_rr/1 -> lamda/9(w_rr)
  lamda/1(lamda_fl) -> lamda_fl/1
  lamda/2(lamda_fr) -> lamda_fr/1
  lamda/4(lamda_rr) -> lamda_rr/1
  lamda/3(lamda_rl) -> lamda_rl/1
  delta_rl/1 -> lamda/10(delta_rl), alpha/6(delta_rl)
  delta_rr/1 -> lamda/11(delta_rr), alpha/7(delta_rr)

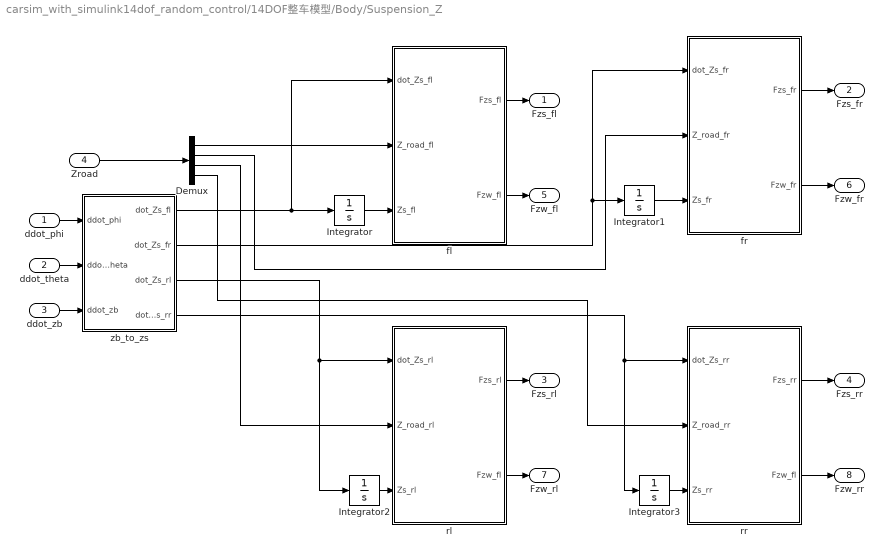
== system carsim_with_simulink14dof_random_control/14DOF整车模型/Body/Suspension_Z ==
  ddot_phi : Inport
  ddot_theta : Inport  Port=2
  ddot_zb : Inport  Port=3
  Zroad : Inport  Port=4
  Demux : Demux
  Integrator{,1..3} (4 alike) : Integrator
  fl : Subsystem
  fr : Subsystem
  rl : Subsystem
  rr : Subsystem
  zb_to_zs : Subsystem
  Fzs_fl : Outport
  Fzs_fr : Outport  Port=2
  Fzs_rl : Outport  Port=3
  Fzs_rr : Outport  Port=4
  Fzw_fl : Outport  Port=5
  Fzw_fr : Outport  Port=6
  Fzw_rl : Outport  Port=7
  Fzw_rr : Outport  Port=8
  wires:
  ddot_phi/1 -> zb_to_zs/1(ddot_phi)
  ddot_theta/1 -> zb_to_zs/2(ddot_theta)
  ddot_zb/1 -> zb_to_zs/3(ddot_zb)
  fl/1(Fzs_fl) -> Fzs_fl/1
  zb_to_zs/1(dot_Zs_fl) -> Integrator/1, fl/1(dot_Zs_fl)
  Zroad/1 -> Demux/1
  Integrator/1 -> fl/3(Zs_fl)
  fr/1(Fzs_fr) -> Fzs_fr/1
  zb_to_zs/2(dot_Zs_fr) -> fr/1(dot_Zs_fr), Integrator1/1
  Demux/2 -> fr/2(Z_road_fr)
  Integrator1/1 -> fr/3(Zs_fr)
  fl/2(Fzw_fl) -> Fzw_fl/1
  fr/2(Fzw_fr) -> Fzw_fr/1
  zb_to_zs/3(dot_Zs_rl) -> rl/1(dot_Zs_rl), Integrator2/1
  Integrator2/1 -> rl/3(Zs_rl)
  Demux/3 -> rl/2(Z_road_rl)
  rl/1(Fzs_rl) -> Fzs_rl/1
  rl/2(Fzw_fl) -> Fzw_rl/1
  zb_to_zs/4(dot_Zs_rr) -> Integrator3/1, rr/1(dot_Zs_rr)
  Demux/4 -> rr/2(Z_road_rr)
  Integrator3/1 -> rr/3(Zs_rr)
  rr/1(Fzs_rr) -> Fzs_rr/1
  rr/2(Fzw_fl) -> Fzw_rr/1
  Demux/1 -> fl/2(Z_road_fl)

== system carsim_with_simulink14dof_random_control/14DOF整车模型/Body/global system transform ==
  vx : Inport
  vy : Inport  Port=2
  wz : Inport  Port=3
  Add : Sum  Inputs=|+-
  Add1 : Sum  Inputs=|++
  Integrator10 : Integrator
  Integrator8 : Integrator
  Integrator9 : Integrator
  Trigonometric Function1 : Trigonometry
  Trigonometric Function2 : Trigonometry  Operator=cos
  vx*cosr : Product
  vx*sinr : Product
  vy*cosr : Product
  vy*sinr : Product
  x : Outport
  y : Outport  Port=2
  wires:
  Add/1 -> Integrator10/1
  Trigonometric Function2/1 -> vy*cosr/2, vx*cosr/2
  vy*sinr/1 -> Add/2
  vx/1 -> vx*sinr/1, vx*cosr/1
  wz/1 -> Integrator8/1
  vy/1 -> vy*sinr/1, vy*cosr/1
  Integrator9/1 -> y/1
  Integrator10/1 -> x/1
  Integrator8/1 -> Trigonometric Function2/1, Trigonometric Function1/1  "r"
  Trigonometric Function1/1 -> vx*sinr/2, vy*sinr/2
  vx*cosr/1 -> Add/1
  vx*sinr/1 -> Add1/1
  Add1/1 -> Integrator9/1
  vy*cosr/1 -> Add1/2

== system carsim_with_simulink14dof_random_control/14DOF整车模型/Wheel/fl ==
  T_fl : Inport
  Fx_fl : Inport  Port=2
  Fz_fl : Inport  Port=3
  Add : Sum  Inputs=+--
  Constant : Constant  Value=I_tire
  Divide : Product  Inputs=*/
  Gain : Gain  Gain=r
  Gain1 : Gain  Gain=r*f
  Integrator : Integrator  InitialCondition=w0
  w_fl : Outport
  wires:
  Integrator/1 -> w_fl/1
  Divide/1 -> Integrator/1  "dot_w"
  Constant/1 -> Divide/2
  Add/1 -> Divide/1
  Gain1/1 -> Add/3
  T_fl/1 -> Add/1
  Fz_fl/1 -> Gain1/1
  Fx_fl/1 -> Gain/1
  Gain/1 -> Add/2

== system carsim_with_simulink14dof_random_control/14DOF整车模型/Wheel/fr ==
  T_fr : Inport
  Fx_fr : Inport  Port=2
  Fz_fr : Inport  Port=3
  Add : Sum  Inputs=+--
  Constant : Constant  Value=I_tire
  Divide : Product  Inputs=*/
  Gain : Gain  Gain=r
  Gain1 : Gain  Gain=r*f
  Integrator : Integrator  InitialCondition=w0
  w_fr : Outport
  wires:
  Fx_fr/1 -> Gain/1
  Fz_fr/1 -> Gain1/1
  T_fr/1 -> Add/1
  Gain/1 -> Add/2
  Add/1 -> Divide/1
  Constant/1 -> Divide/2
  Divide/1 -> Integrator/1  "dot_w"
  Integrator/1 -> w_fr/1
  Gain1/1 -> Add/3

== system carsim_with_simulink14dof_random_control/14DOF整车模型/Wheel/rl ==
  T_rl : Inport
  Fx_rl : Inport  Port=2
  Fz_rl : Inport  Port=3
  Add : Sum  Inputs=+--
  Constant : Constant  Value=I_tire
  Divide : Product  Inputs=*/
  Gain : Gain  Gain=r
  Gain1 : Gain  Gain=r*f
  Integrator : Integrator  InitialCondition=w0
  w_rl : Outport
  wires:
  Fx_rl/1 -> Gain/1
  Fz_rl/1 -> Gain1/1
  T_rl/1 -> Add/1
  Gain/1 -> Add/2
  Add/1 -> Divide/1
  Constant/1 -> Divide/2
  Divide/1 -> Integrator/1  "dot_w"
  Integrator/1 -> w_rl/1
  Gain1/1 -> Add/3

== system carsim_with_simulink14dof_random_control/14DOF整车模型/Wheel/rr ==
  T_rr : Inport
  Fx_rr : Inport  Port=2
  Fz_rr : Inport  Port=3
  Add : Sum  Inputs=+--
  Constant : Constant  Value=I_tire
  Divide : Product  Inputs=*/
  Gain : Gain  Gain=r
  Gain1 : Gain  Gain=r*f
  Integrator : Integrator  InitialCondition=w0
  w_rr : Outport
  wires:
  Integrator/1 -> w_rr/1
  Divide/1 -> Integrator/1  "dot_w"
  Constant/1 -> Divide/2
  Add/1 -> Divide/1
  Gain/1 -> Add/2
  T_rr/1 -> Add/1
  Fz_rr/1 -> Gain1/1
  Fx_rr/1 -> Gain/1
  Gain1/1 -> Add/3

== system carsim_with_simulink14dof_random_control/14DOF整车模型/alpha_lamda/alpha ==
  vx : Inport
  vy : Inport  Port=2
  wz : Inport  Port=3
  delta_fl : Inport  Port=4
  delta_fr : Inport  Port=5
  delta_rl : Inport  Port=6
  delta_rr : Inport  Port=7
  Gain{,1..3} (4 alike) : Gain  Gain=-1
  fl : Subsystem
  fr : Subsystem
  rl : Subsystem
  rr : Subsystem
  alpha_fl : Outport
  alpha_fr : Outport  Port=2
  alpha_rl : Outport  Port=3
  alpha_rr : Outport  Port=4
  wires:
  Gain3/1 -> alpha_rr/1
  rr/1(alpha_rr) -> Gain3/1
  Gain2/1 -> alpha_fr/1
  fr/1(alpha_fr) -> Gain2/1
  Gain1/1 -> alpha_rl/1
  rl/1(alpha_rl) -> Gain1/1
  Gain/1 -> alpha_fl/1
  fl/1(alpha_fl) -> Gain/1
  wz/1 -> fl/3(wz), rr/3(wz), fr/3(wz), rl/3(wz)
  vx/1 -> rr/1(vx), fr/1(vx), fl/1(vx), rl/1(vx)
  vy/1 -> rr/2(vy), fr/2(vy), fl/2(vy), rl/2(vy)
  delta_fl/1 -> fl/4(delta_fl)
  delta_fr/1 -> fr/4(delta_fr)
  delta_rl/1 -> rl/4(delta_rl)
  delta_rr/1 -> rr/4(delta_rr)

== system carsim_with_simulink14dof_random_control/14DOF整车模型/alpha_lamda/lamda ==
  vx : Inport
  vy : Inport  Port=2
  wz : Inport  Port=3
  delta_fl : Inport  Port=4
  delta_fr : Inport  Port=5
  w_fl : Inport  Port=6
  w_fr : Inport  Port=7
  w_rl : Inport  Port=8
  w_rr : Inport  Port=9
  delta_rl : Inport  Port=10
  delta_rr : Inport  Port=11
  fl : Subsystem
  fr : Subsystem
  rl : Subsystem
  rr : Subsystem
  lamda_fl : Outport
  lamda_fr : Outport  Port=2
  lamda_rl : Outport  Port=3
  lamda_rr : Outport  Port=4
  wires:
  fl/1(lamda_fl) -> lamda_fl/1
  rl/1(lamda_rl) -> lamda_rl/1
  w_fl/1 -> fl/1(w_fl)
  wz/1 -> rl/2(wz), rr/2(wz), fr/2(wz), fl/2(wz)
  vx/1 -> rl/3(vx), rr/3(vx), fr/3(vx), fl/3(vx)
  vy/1 -> rl/4(vy), rr/4(vy), fr/4(vy), fl/4(vy)
  delta_fl/1 -> fl/5(delta_fl)
  delta_fr/1 -> fr/5(delta_fr)
  w_fr/1 -> fr/1(w_fr)
  w_rr/1 -> rr/1(w_rr)
  w_rl/1 -> rl/1(w_rl)
  rr/1(lamda_rr) -> lamda_rr/1
  fr/1(lamda_fr) -> lamda_fr/1
  delta_rl/1 -> rl/5(delta_rl)
  delta_rr/1 -> rr/5(delta_rr)

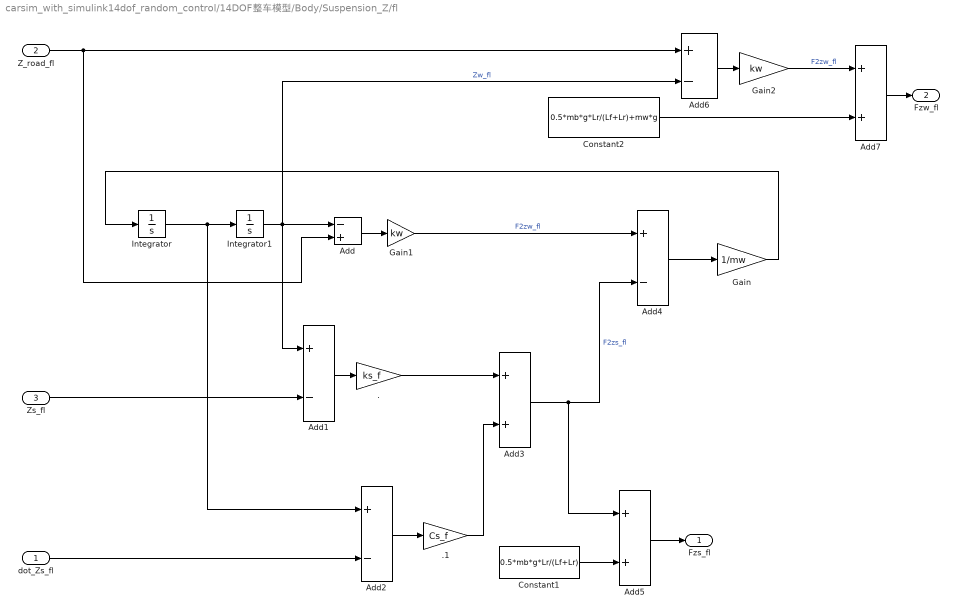
== system carsim_with_simulink14dof_random_control/14DOF整车模型/Body/Suspension_Z/fl ==
  dot_Zs_fl : Inport
  Z_road_fl : Inport  Port=2
  Zs_fl : Inport  Port=3
  . : Gain  Gain=ks_f
  .1 : Gain  Gain=Cs_f
  Add : Sum  Inputs=-+
  Add{1..2,4,6} (4 alike) : Sum  Inputs=+-
  Add3 : Sum
  Add5 : Sum
  Add7 : Sum
  Constant1 : Constant  Value=0.5*mb*g*Lr/(Lf+Lr)
  Constant2 : Constant  Value=0.5*mb*g*Lr/(Lf+Lr)+mw*g
  Gain : Gain  Gain=1/mw
  Gain1 : Gain  Gain=kw
  Gain2 : Gain  Gain=kw
  Integrator : Integrator
  Integrator1 : Integrator
  Fzs_fl : Outport
  Fzw_fl : Outport  Port=2
  wires:
  Add5/1 -> Fzs_fl/1
  Constant1/1 -> Add5/2
  Integrator/1 -> Add2/1, Integrator1/1
  Integrator1/1 -> Add6/2, Add1/1, Add/1  "Zw_fl"
  Z_road_fl/1 -> Add/2, Add6/1
  Add/1 -> Gain1/1
  Gain1/1 -> Add4/1  "F2zw_fl"
  Zs_fl/1 -> Add1/2
  Add1/1 -> ./1
  dot_Zs_fl/1 -> Add2/2
  Add2/1 -> .1/1
  ./1 -> Add3/1
  .1/1 -> Add3/2
  Add3/1 -> Add4/2, Add5/1  "F2zs_fl"
  Add4/1 -> Gain/1
  Gain/1 -> Integrator/1
  Add6/1 -> Gain2/1
  Gain2/1 -> Add7/1  "F2zw_fl"
  Constant2/1 -> Add7/2
  Add7/1 -> Fzw_fl/1

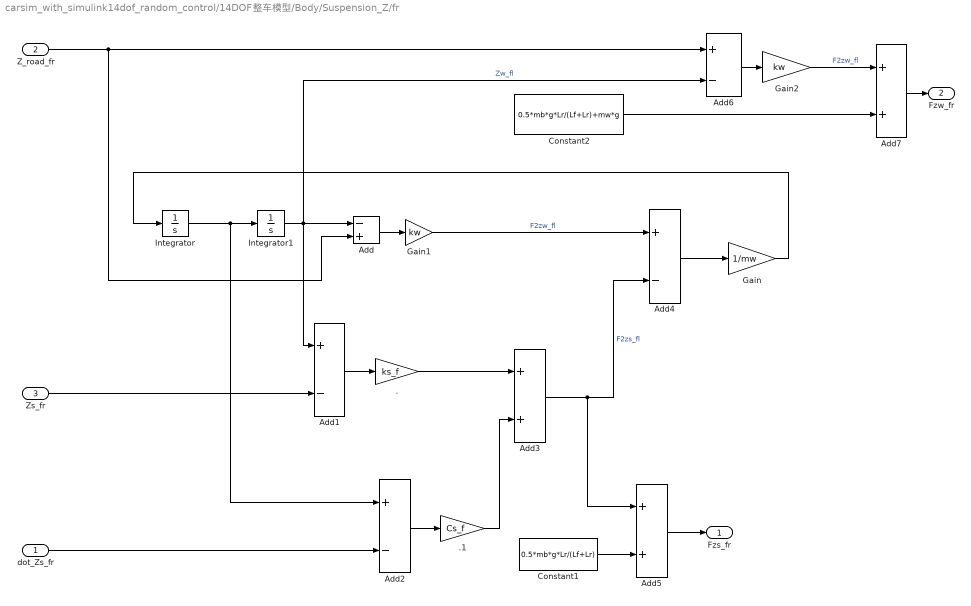
== system carsim_with_simulink14dof_random_control/14DOF整车模型/Body/Suspension_Z/fr ==
  dot_Zs_fr : Inport
  Z_road_fr : Inport  Port=2
  Zs_fr : Inport  Port=3
  . : Gain  Gain=ks_f
  .1 : Gain  Gain=Cs_f
  Add : Sum  Inputs=-+
  Add{1..2,4,6} (4 alike) : Sum  Inputs=+-
  Add3 : Sum
  Add5 : Sum
  Add7 : Sum
  Constant1 : Constant  Value=0.5*mb*g*Lr/(Lf+Lr)
  Constant2 : Constant  Value=0.5*mb*g*Lr/(Lf+Lr)+mw*g
  Gain : Gain  Gain=1/mw
  Gain1 : Gain  Gain=kw
  Gain2 : Gain  Gain=kw
  Integrator : Integrator
  Integrator1 : Integrator
  Fzs_fr : Outport
  Fzw_fr : Outport  Port=2
  wires:
  Add5/1 -> Fzs_fr/1
  Constant1/1 -> Add5/2
  Add3/1 -> Add4/2, Add5/1  "F2zs_fl"
  Gain/1 -> Integrator/1
  Add4/1 -> Gain/1
  .1/1 -> Add3/2
  ./1 -> Add3/1
  Add2/1 -> .1/1
  dot_Zs_fr/1 -> Add2/2
  Add1/1 -> ./1
  Zs_fr/1 -> Add1/2
  Add/1 -> Gain1/1
  Integrator1/1 -> Add/1, Add1/1, Add6/2  "Zw_fl"
  Integrator/1 -> Integrator1/1, Add2/1
  Z_road_fr/1 -> Add6/1, Add/2
  Gain1/1 -> Add4/1  "F2zw_fl"
  Add6/1 -> Gain2/1
  Gain2/1 -> Add7/1  "F2zw_fl"
  Constant2/1 -> Add7/2
  Add7/1 -> Fzw_fr/1

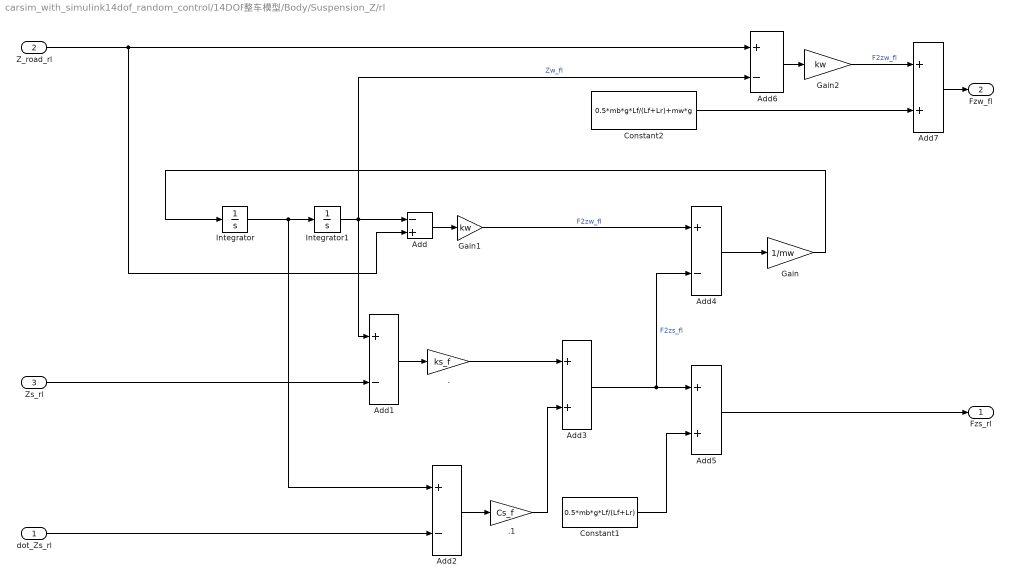
== system carsim_with_simulink14dof_random_control/14DOF整车模型/Body/Suspension_Z/rl ==
  dot_Zs_rl : Inport
  Z_road_rl : Inport  Port=2
  Zs_rl : Inport  Port=3
  . : Gain  Gain=ks_f
  .1 : Gain  Gain=Cs_f
  Add : Sum  Inputs=-+
  Add{1..2,4,6} (4 alike) : Sum  Inputs=+-
  Add3 : Sum
  Add5 : Sum
  Add7 : Sum
  Constant1 : Constant  Value=0.5*mb*g*Lf/(Lf+Lr)
  Constant2 : Constant  Value=0.5*mb*g*Lf/(Lf+Lr)+mw*g
  Gain : Gain  Gain=1/mw
  Gain1 : Gain  Gain=kw
  Gain2 : Gain  Gain=kw
  Integrator : Integrator
  Integrator1 : Integrator
  Fzs_rl : Outport
  Fzw_fl : Outport  Port=2
  wires:
  Add5/1 -> Fzs_rl/1
  Constant1/1 -> Add5/2
  Add3/1 -> Add4/2, Add5/1  "F2zs_fl"
  Gain/1 -> Integrator/1
  Add4/1 -> Gain/1
  .1/1 -> Add3/2
  ./1 -> Add3/1
  Add2/1 -> .1/1
  dot_Zs_rl/1 -> Add2/2
  Add1/1 -> ./1
  Zs_rl/1 -> Add1/2
  Add/1 -> Gain1/1
  Integrator1/1 -> Add/1, Add1/1, Add6/2  "Zw_fl"
  Integrator/1 -> Integrator1/1, Add2/1
  Z_road_rl/1 -> Add6/1, Add/2
  Gain1/1 -> Add4/1  "F2zw_fl"
  Add6/1 -> Gain2/1
  Gain2/1 -> Add7/1  "F2zw_fl"
  Constant2/1 -> Add7/2
  Add7/1 -> Fzw_fl/1

== system carsim_with_simulink14dof_random_control/14DOF整车模型/Body/Suspension_Z/rr ==
  dot_Zs_rr : Inport
  Z_road_rr : Inport  Port=2
  Zs_rr : Inport  Port=3
  . : Gain  Gain=ks_f
  .1 : Gain  Gain=Cs_f
  Add : Sum  Inputs=-+
  Add{1..2,4,6} (4 alike) : Sum  Inputs=+-
  Add3 : Sum
  Add5 : Sum
  Add7 : Sum
  Constant1 : Constant  Value=0.5*mb*g*Lf/(Lf+Lr)
  Constant2 : Constant  Value=0.5*mb*g*Lf/(Lf+Lr)+mw*g
  Gain : Gain  Gain=1/mw
  Gain1 : Gain  Gain=kw
  Gain2 : Gain  Gain=kw
  Integrator : Integrator
  Integrator1 : Integrator
  Fzs_rr : Outport
  Fzw_fl : Outport  Port=2
  wires:
  Add5/1 -> Fzs_rr/1
  Constant1/1 -> Add5/2
  Add3/1 -> Add4/2, Add5/1  "F2zs_fl"
  Integrator/1 -> Add2/1, Integrator1/1
  Integrator1/1 -> Add6/2, Add1/1, Add/1  "Zw_fl"
  Add/1 -> Gain1/1
  Zs_rr/1 -> Add1/2
  Add1/1 -> ./1
  dot_Zs_rr/1 -> Add2/2
  Add2/1 -> .1/1
  ./1 -> Add3/1
  .1/1 -> Add3/2
  Add4/1 -> Gain/1
  Gain/1 -> Integrator/1
  Z_road_rr/1 -> Add6/1, Add/2
  Gain1/1 -> Add4/1  "F2zw_fl"
  Add6/1 -> Gain2/1
  Gain2/1 -> Add7/1  "F2zw_fl"
  Constant2/1 -> Add7/2
  Add7/1 -> Fzw_fl/1

== system carsim_with_simulink14dof_random_control/14DOF整车模型/Body/Suspension_Z/zb_to_zs ==
  ddot_phi : Inport
  ddot_theta : Inport  Port=2
  ddot_zb : Inport  Port=3
  Bf/2 : Gain  Gain=0.5*Bf
  Br/2 : Gain  Gain=0.5*Br
  Integrator{,1..3} (4 alike) : Integrator
  Lf : Gain  Gain=Lf
  Lr : Gain  Gain=Lr
  Sum1 : Sum  Inputs=+--
  Sum2 : Sum  Inputs=+++
  Sum3 : Sum  Inputs=+-+
  Sum8 : Sum  Inputs=++-
  dot_Zs_fl : Outport
  dot_Zs_fr : Outport  Port=2
  dot_Zs_rl : Outport  Port=3
  dot_Zs_rr : Outport  Port=4
  wires:
  ddot_phi/1 -> Br/2/1, Bf/2/1
  ddot_theta/1 -> Lr/1, Lf/1
  ddot_zb/1 -> Sum8/1, Sum1/1, Sum3/1, Sum2/1
  Bf/2/1 -> Sum1/2, Sum8/2
  Lf/1 -> Sum1/3, Sum8/3
  Sum8/1 -> Integrator/1
  Sum1/1 -> Integrator1/1
  Br/2/1 -> Sum3/2, Sum2/2
  Lr/1 -> Sum3/3, Sum2/3
  Sum2/1 -> Integrator2/1
  Sum3/1 -> Integrator3/1
  Integrator/1 -> dot_Zs_fl/1
  Integrator1/1 -> dot_Zs_fr/1
  Integrator2/1 -> dot_Zs_rl/1
  Integrator3/1 -> dot_Zs_rr/1

== system carsim_with_simulink14dof_random_control/14DOF整车模型/alpha_lamda/alpha/fl ==
  vx : Inport
  vy : Inport  Port=2
  wz : Inport  Port=3
  delta_fl : Inport  Port=4
  Add2 : Sum
  Add3 : Sum  Inputs=+-
  Add4 : Sum  Inputs=-+
  Divide : Product  Inputs=/*
  Gain3 : Gain  Gain=Lf
  Gain4 : Gain  Gain=0.5*Bf
  Scope : Scope
  Trigonometric Function : Trigonometry  Operator=atan
  alpha_fl : Outport
  wires:
  Gain3/1 -> Add2/2
  Gain4/1 -> Add3/2
  Add2/1 -> Divide/2
  Add3/1 -> Divide/1
  Divide/1 -> Trigonometric Function/1
  Trigonometric Function/1 -> Scope/1, Add4/1
  vx/1 -> Add3/1
  delta_fl/1 -> Add4/2
  vy/1 -> Add2/1
  Add4/1 -> alpha_fl/1
  wz/1 -> Gain4/1, Gain3/1

== system carsim_with_simulink14dof_random_control/14DOF整车模型/alpha_lamda/alpha/fr ==
  vx : Inport
  vy : Inport  Port=2
  wz : Inport  Port=3
  delta_fr : Inport  Port=4
  Add2 : Sum
  Add3 : Sum
  Add4 : Sum  Inputs=-+
  Divide : Product  Inputs=/*
  Gain3 : Gain  Gain=Lf
  Gain4 : Gain  Gain=0.5*Bf
  Trigonometric Function : Trigonometry  Operator=atan
  alpha_fr : Outport
  wires:
  Gain4/1 -> Add3/2
  wz/1 -> Gain3/1, Gain4/1
  Add4/1 -> alpha_fr/1
  vy/1 -> Add2/1
  delta_fr/1 -> Add4/2
  vx/1 -> Add3/1
  Trigonometric Function/1 -> Add4/1
  Divide/1 -> Trigonometric Function/1
  Add3/1 -> Divide/1
  Add2/1 -> Divide/2
  Gain3/1 -> Add2/2

== system carsim_with_simulink14dof_random_control/14DOF整车模型/alpha_lamda/alpha/rl ==
  vx : Inport
  vy : Inport  Port=2
  wz : Inport  Port=3
  delta_rl : Inport  Port=4
  Add2 : Sum  Inputs=+-
  Add3 : Sum  Inputs=+-
  Add4 : Sum  Inputs=-+
  Divide : Product  Inputs=/*
  Gain3 : Gain  Gain=Lr
  Gain4 : Gain  Gain=0.5*Br
  Trigonometric Function : Trigonometry  Operator=atan
  alpha_rl : Outport
  wires:
  Add4/1 -> alpha_rl/1
  Gain4/1 -> Add3/2
  Trigonometric Function/1 -> Add4/1
  wz/1 -> Gain3/1, Gain4/1  "wz"
  vy/1 -> Add2/1  "vy"
  vx/1 -> Add3/1  "vx"
  Divide/1 -> Trigonometric Function/1
  Add3/1 -> Divide/1  "Vx_rl"
  Add2/1 -> Divide/2  "Vy_rl"
  Gain3/1 -> Add2/2
  delta_rl/1 -> Add4/2

== system carsim_with_simulink14dof_random_control/14DOF整车模型/alpha_lamda/alpha/rr ==
  vx : Inport
  vy : Inport  Port=2
  wz : Inport  Port=3
  delta_rr : Inport  Port=4
  Add2 : Sum  Inputs=+-
  Add3 : Sum
  Add4 : Sum  Inputs=-+
  Divide : Product  Inputs=/*
  Gain3 : Gain  Gain=Lr
  Gain4 : Gain  Gain=0.5*Br
  Trigonometric Function : Trigonometry  Operator=atan
  alpha_rr : Outport
  wires:
  Add4/1 -> alpha_rr/1
  Gain4/1 -> Add3/2
  Gain3/1 -> Add2/2
  Add2/1 -> Divide/2  "Vy_rr"
  Add3/1 -> Divide/1  "Vx_rr"
  Divide/1 -> Trigonometric Function/1
  vx/1 -> Add3/1  "vx"
  vy/1 -> Add2/1  "vy"
  wz/1 -> Gain4/1, Gain3/1  "wz"
  Trigonometric Function/1 -> Add4/1
  delta_rr/1 -> Add4/2

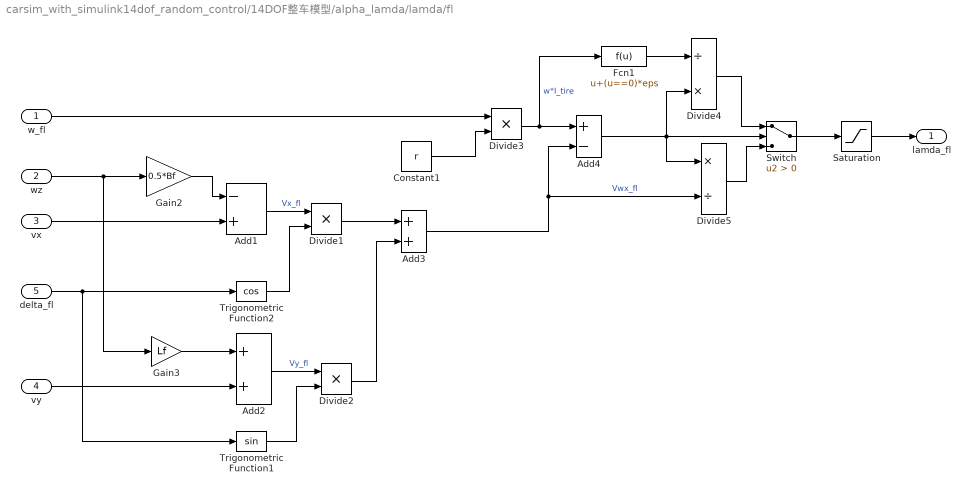
== system carsim_with_simulink14dof_random_control/14DOF整车模型/alpha_lamda/lamda/fl ==
  w_fl : Inport
  wz : Inport  Port=2
  vx : Inport  Port=3
  vy : Inport  Port=4
  delta_fl : Inport  Port=5
  Add1 : Sum  Inputs=-+
  Add2 : Sum
  Add3 : Sum
  Add4 : Sum  Inputs=+-
  Constant1 : Constant  Value=r
  Divide1 : Product  Inputs=**
  Divide2 : Product  Inputs=**
  Divide3 : Product  Inputs=**
  Divide4 : Product  Inputs=/*
  Divide5 : Product  Inputs=*/
  Fcn1 : Fcn  Expr=u+(u==0)*eps
  Gain2 : Gain  Gain=0.5*Bf
  Gain3 : Gain  Gain=Lf
  Saturation : Saturate  UpperLimit=1  LowerLimit=-1
  Switch : Switch  Criteria=u2 > Threshold  SaturateOnIntegerOverflow=off  InputSameDT=off
  Trigonometric Function1 : Trigonometry
  Trigonometric Function2 : Trigonometry  Operator=cos
  lamda_fl : Outport
  wires:
  Saturation/1 -> lamda_fl/1
  Divide3/1 -> Fcn1/1, Add4/1  "w*I_tire"
  Constant1/1 -> Divide3/2
  w_fl/1 -> Divide3/1
  Divide2/1 -> Add3/2
  Divide1/1 -> Add3/1
  Trigonometric Function1/1 -> Divide2/2
  Add2/1 -> Divide2/1  "Vy_fl"
  Gain3/1 -> Add2/1
  vy/1 -> Add2/2
  Trigonometric Function2/1 -> Divide1/2
  delta_fl/1 -> Trigonometric Function1/1, Trigonometric Function2/1
  Add1/1 -> Divide1/1  "Vx_fl"
  wz/1 -> Gain2/1, Gain3/1
  Gain2/1 -> Add1/1
  vx/1 -> Add1/2
  Fcn1/1 -> Divide4/1
  Divide5/1 -> Switch/3
  Divide4/1 -> Switch/1
  Add4/1 -> Divide5/1, Divide4/2, Switch/2
  Add3/1 -> Divide5/2, Add4/2  "Vwx_fl"
  Switch/1 -> Saturation/1

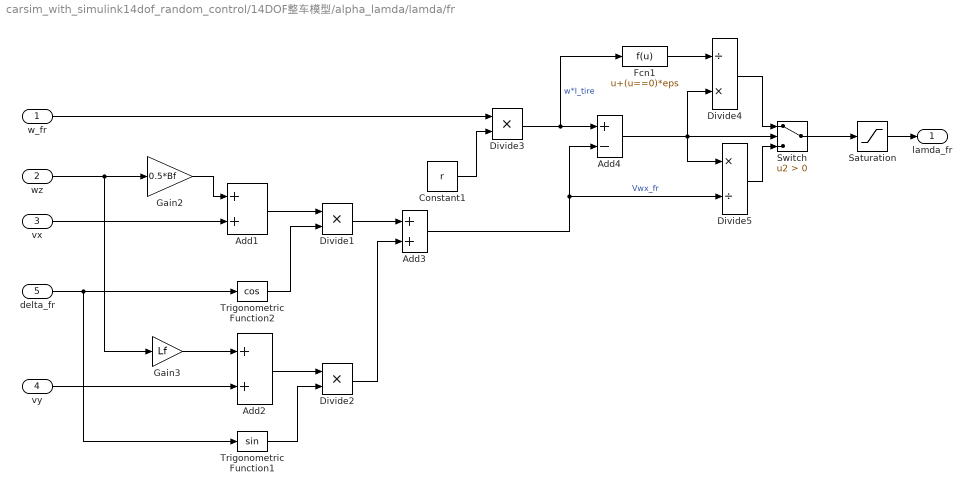
== system carsim_with_simulink14dof_random_control/14DOF整车模型/alpha_lamda/lamda/fr ==
  w_fr : Inport
  wz : Inport  Port=2
  vx : Inport  Port=3
  vy : Inport  Port=4
  delta_fr : Inport  Port=5
  Add1 : Sum
  Add2 : Sum
  Add3 : Sum
  Add4 : Sum  Inputs=+-
  Constant1 : Constant  Value=r
  Divide1 : Product  Inputs=**
  Divide2 : Product  Inputs=**
  Divide3 : Product  Inputs=**
  Divide4 : Product  Inputs=/*
  Divide5 : Product  Inputs=*/
  Fcn1 : Fcn  Expr=u+(u==0)*eps
  Gain2 : Gain  Gain=0.5*Bf
  Gain3 : Gain  Gain=Lf
  Saturation : Saturate  UpperLimit=1  LowerLimit=-1
  Switch : Switch  Criteria=u2 > Threshold  SaturateOnIntegerOverflow=off  InputSameDT=off
  Trigonometric Function1 : Trigonometry
  Trigonometric Function2 : Trigonometry  Operator=cos
  lamda_fr : Outport
  wires:
  Switch/1 -> Saturation/1
  Add3/1 -> Add4/2, Divide5/2  "Vwx_fr"
  Add4/1 -> Switch/2, Divide4/2, Divide5/1
  Divide4/1 -> Switch/1
  Divide5/1 -> Switch/3
  Fcn1/1 -> Divide4/1
  Divide3/1 -> Add4/1, Fcn1/1  "w*I_tire"
  Constant1/1 -> Divide3/2
  w_fr/1 -> Divide3/1
  Divide2/1 -> Add3/2
  Divide1/1 -> Add3/1
  Trigonometric Function1/1 -> Divide2/2
  Add2/1 -> Divide2/1
  Gain3/1 -> Add2/1
  vy/1 -> Add2/2
  Trigonometric Function2/1 -> Divide1/2
  delta_fr/1 -> Trigonometric Function1/1, Trigonometric Function2/1
  Add1/1 -> Divide1/1
  wz/1 -> Gain2/1, Gain3/1
  Gain2/1 -> Add1/1
  vx/1 -> Add1/2
  Saturation/1 -> lamda_fr/1

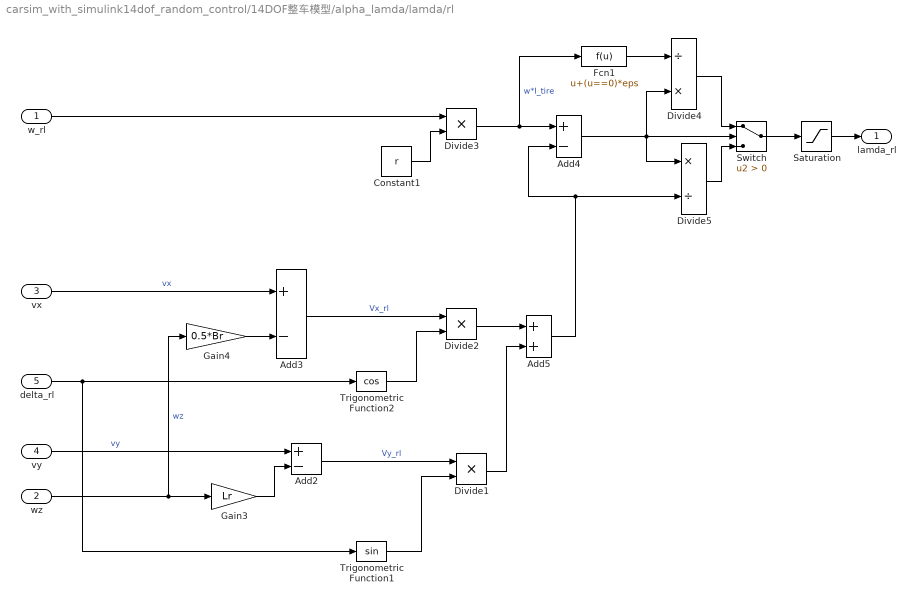
== system carsim_with_simulink14dof_random_control/14DOF整车模型/alpha_lamda/lamda/rl ==
  w_rl : Inport
  wz : Inport  Port=2
  vx : Inport  Port=3
  vy : Inport  Port=4
  delta_rl : Inport  Port=5
  Add2 : Sum  Inputs=+-
  Add3 : Sum  Inputs=+-
  Add4 : Sum  Inputs=+-
  Add5 : Sum
  Constant1 : Constant  Value=r
  Divide1 : Product  Inputs=**
  Divide2 : Product  Inputs=**
  Divide3 : Product  Inputs=**
  Divide4 : Product  Inputs=/*
  Divide5 : Product  Inputs=*/
  Fcn1 : Fcn  Expr=u+(u==0)*eps
  Gain3 : Gain  Gain=Lr
  Gain4 : Gain  Gain=0.5*Br
  Saturation : Saturate  UpperLimit=1  LowerLimit=-1
  Switch : Switch  Criteria=u2 > Threshold  SaturateOnIntegerOverflow=off  InputSameDT=off
  Trigonometric Function1 : Trigonometry
  Trigonometric Function2 : Trigonometry  Operator=cos
  lamda_rl : Outport
  wires:
  Switch/1 -> Saturation/1
  Add4/1 -> Switch/2, Divide4/2, Divide5/1
  Divide4/1 -> Switch/1
  Divide5/1 -> Switch/3
  Fcn1/1 -> Divide4/1
  Divide3/1 -> Add4/1, Fcn1/1  "w*I_tire"
  Constant1/1 -> Divide3/2
  w_rl/1 -> Divide3/1
  Saturation/1 -> lamda_rl/1
  Gain4/1 -> Add3/2
  wz/1 -> Gain3/1, Gain4/1  "wz"
  vy/1 -> Add2/1  "vy"
  vx/1 -> Add3/1  "vx"
  Add3/1 -> Divide2/1  "Vx_rl"
  Add2/1 -> Divide1/1  "Vy_rl"
  Gain3/1 -> Add2/2
  delta_rl/1 -> Trigonometric Function1/1, Trigonometric Function2/1
  Trigonometric Function2/1 -> Divide2/2
  Divide2/1 -> Add5/1
  Trigonometric Function1/1 -> Divide1/2
  Divide1/1 -> Add5/2
  Add5/1 -> Add4/2, Divide5/2

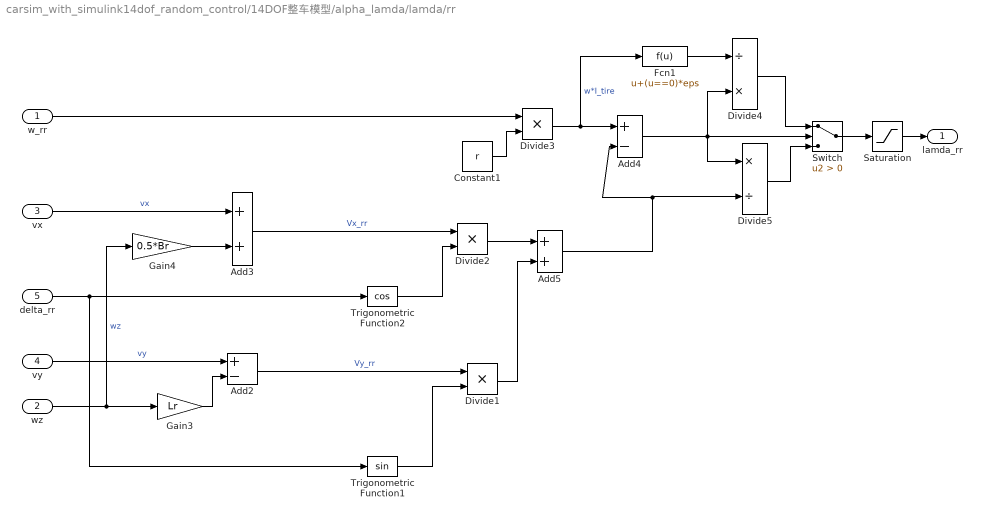
== system carsim_with_simulink14dof_random_control/14DOF整车模型/alpha_lamda/lamda/rr ==
  w_rr : Inport
  wz : Inport  Port=2
  vx : Inport  Port=3
  vy : Inport  Port=4
  delta_rr : Inport  Port=5
  Add2 : Sum  Inputs=+-
  Add3 : Sum
  Add4 : Sum  Inputs=+-
  Add5 : Sum
  Constant1 : Constant  Value=r
  Divide1 : Product  Inputs=**
  Divide2 : Product  Inputs=**
  Divide3 : Product  Inputs=**
  Divide4 : Product  Inputs=/*
  Divide5 : Product  Inputs=*/
  Fcn1 : Fcn  Expr=u+(u==0)*eps
  Gain3 : Gain  Gain=Lr
  Gain4 : Gain  Gain=0.5*Br
  Saturation : Saturate  UpperLimit=1  LowerLimit=-1
  Switch : Switch  Criteria=u2 > Threshold  SaturateOnIntegerOverflow=off  InputSameDT=off
  Trigonometric Function1 : Trigonometry
  Trigonometric Function2 : Trigonometry  Operator=cos
  lamda_rr : Outport
  wires:
  Add4/1 -> Switch/2, Divide4/2, Divide5/1
  Divide4/1 -> Switch/1
  Divide5/1 -> Switch/3
  Fcn1/1 -> Divide4/1
  Divide3/1 -> Add4/1, Fcn1/1  "w*I_tire"
  w_rr/1 -> Divide3/1
  Constant1/1 -> Divide3/2
  Switch/1 -> Saturation/1
  Saturation/1 -> lamda_rr/1
  Gain4/1 -> Add3/2
  Gain3/1 -> Add2/2
  Add2/1 -> Divide1/1  "Vy_rr"
  Add3/1 -> Divide2/1  "Vx_rr"
  vx/1 -> Add3/1  "vx"
  vy/1 -> Add2/1  "vy"
  wz/1 -> Gain4/1, Gain3/1  "wz"
  Trigonometric Function2/1 -> Divide2/2
  Divide2/1 -> Add5/1
  Trigonometric Function1/1 -> Divide1/2
  Divide1/1 -> Add5/2
  delta_rr/1 -> Trigonometric Function1/1, Trigonometric Function2/1
  Add5/1 -> Add4/2, Divide5/2
